simulink model "ecu_boostg"  (R2026a)
settings: Solver=FixedStepDiscrete  StopTime=10  FixedStep=0.001  SampleTimeConstraint=STIndependent
Description:
  | Boost overvoltage guard. Source of truth for firmware/gen/ecu_boostg.
settings Model: Creator=jj1001000  LastModifiedBy=jj1001000
settings OptimizationCC: DefaultUnderspecifiedDataType=single
settings DebuggingCC: ParameterPrecisionLossMsg=none
settings HardwareCC: ProdLargestAtomicInteger=Long  ProdLargestAtomicFloat=Double  ProdHWDeviceType=ARM Compatible->ARM Cortex-M
settings RTWCC: SystemTargetFile=ert.tlc  GenCodeOnly=on  Description=Embedded Coder
settings ERTTargetCC: UtilityFuncGeneration=Shared location  IncludeMdlTerminateFcn=off  CodeInterfacePackaging=Reusable function  SupportNonFinite=off

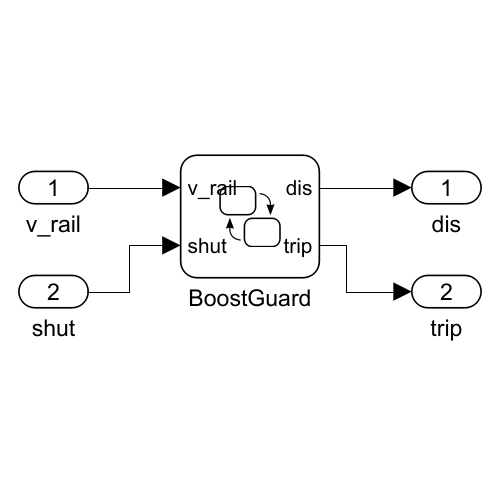
[thumbnail: Simulink's stored preview of the top-level diagram]
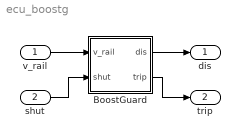
== system ecu_boostg ==
  v_rail : Inport  OutDataTypeStr=single
  shut : Inport  Port=2  OutDataTypeStr=uint8
  BoostGuard : Stateflow chart  TreatAsAtomicUnit=on
  dis : Outport  OutDataTypeStr=uint8
  trip : Outport  Port=2  OutDataTypeStr=uint8
  wires:
  v_rail/1 -> BoostGuard/1(v_rail)
  BoostGuard/2(trip) -> trip/1
  BoostGuard/1(dis) -> dis/1
  shut/1 -> BoostGuard/2(shut)

== stateflow chart ecu_boostg/BoostGuard ==
  settings: updateMethod=DISCRETE  executeAtInitialization=1
  state Guard
    entry: cnt = uint16(0); latched = uint8(0); dis = uint8(0); trip = uint8(0);
    during: trip = uint8(0); dis = uint8(shut ~= 0 || latched ~= 0);
    state OK
    state HIGH
      during: cnt = cnt + 1;
    state LATCHED
      entry: latched = uint8(1); dis = uint8(1);
    (default) -> OK
    OK -> HIGH : [v_rail > single(106)]{cnt = uint16(1);}
    HIGH -> LATCHED [order 2] : [cnt + 1 >= uint16(20)]{trip = uint8(1);}
    HIGH -> OK [order 1] : [v_rail <= single(106)]
  (default) -> Guard
  data: v_rail input single; shut input uint8; dis output uint8; trip output uint8; cnt local uint16; latched local uint8
